simulink model "WSLS_X_Y_Rz3"  (R2025a)
settings: Solver=FixedStepAuto  StartTime=0.0  StopTime=t_end  FixedStep=0.0002  RelTol=1e-3  EnableMultiTasking=on
values from neighbouring files (symbols this model uses):
  rzQ = mz/k    (= 4.2809)    [Multiple_main_Control.m]
  Tb = pinv(B1)    [Multiple_main_Control.m]
  Ty = pinv(C1)    [Multiple_main_Control.m]
  xQ = Jrx/k    (= 0.0439)    [Multiple_main_Control.m]
  yQ = Jry/k    (= 0.0384)    [Multiple_main_Control.m]
undefined symbols (not defined in the file or in its folder): den_Cfb_rz, den_Cfb_x, den_Cfb_y, den_P11, den_P12, den_P13, den_P14, den_P21, den_P22, den_P23, den_P24, den_P31, den_P32, den_P33, den_P34, den_P41, den_P42, den_P43, den_P44, num_Cfb_rz, num_Cfb_x, num_Cfb_y, num_P11, num_P12, num_P13, num_P14, num_P21, num_P22, num_P23, num_P24, num_P31, num_P32, num_P33, num_P34, num_P41, num_P42, num_P43, num_P44
settings Model: Creator=zhang chen  LastModifiedBy=gdc24
settings DataIOCC: ReturnWorkspaceOutputs=off
settings OptimizationCC: ReuseModelBlockBuffer=off
settings DebuggingCC: UnconnectedInputMsg=warning  UnconnectedOutputMsg=warning  UnconnectedLineMsg=warning
settings ModelReferenceCC: EnableRefExpFcnMdlSchedulingChecks=on
settings RTWCC: GPUComputeCapability=3.5  DLArmComputeVersion=19.05

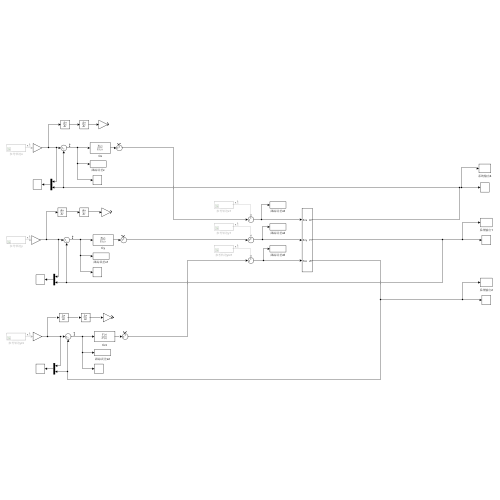
[thumbnail: Simulink's stored preview of the top-level diagram]
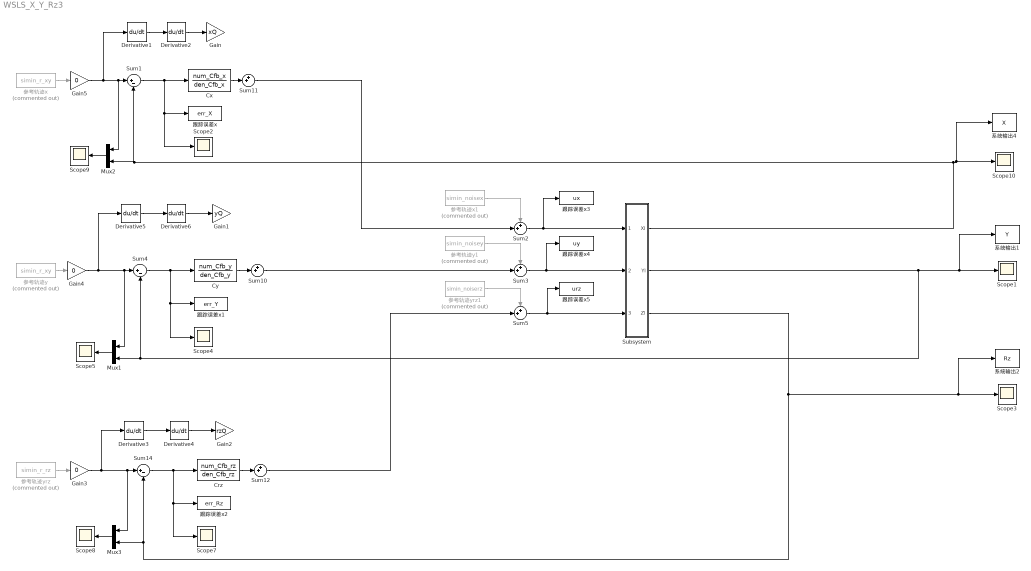
== system WSLS_X_Y_Rz3 ==
  Crz : TransferFcn  Numerator=num_Cfb_rz  Denominator=den_Cfb_rz
  Cx : TransferFcn  Numerator=num_Cfb_x  Denominator=den_Cfb_x
  Cy : TransferFcn  Numerator=num_Cfb_y  Denominator=den_Cfb_y
  Derivative{1..6} (6 alike) : Derivative
  Gain : Gain  Gain=xQ
  Gain1 : Gain  Gain=yQ
  Gain2 : Gain  Gain=rzQ
  Gain3 : Gain  Gain=0
  Gain4 : Gain  Gain=0
  Gain5 : Gain  Gain=0
  Mux1 : Mux  Inputs=2
  Mux2 : Mux  Inputs=2
  Mux3 : Mux  Inputs=2
  Scope{1..5,7..10} (9 alike) : Scope
      Scope1 settings: ActiveDisplayYMinimum=-8.79901930835965E-7  ActiveDisplayYMaximum=1.0139843335391608E-6  DataLoggingVariableName=ScopeData2
      Scope10 settings: ActiveDisplayYMinimum=-5.7566992518821054E-6  ActiveDisplayYMaximum=3.1982882643224368E-6
      Scope2 settings: ActiveDisplayYMinimum=-9E-7  ActiveDisplayYMaximum=9E-7
      Scope3 settings: ActiveDisplayYMinimum=-2.3040708038382956E-6  ActiveDisplayYMaximum=2.1091467969503966E-6  DataLoggingVariableName=ScopeData3
      Scope4 settings: ActiveDisplayYMinimum=-5E-7  ActiveDisplayYMaximum=6E-7  DataLoggingVariableName=ScopeData4
      Scope5 settings: ActiveDisplayYMinimum=-0.225  ActiveDisplayYMaximum=0.025  DataLoggingVariableName=ScopeData5
      Scope7 settings: ActiveDisplayYMinimum=-3.8E-5  ActiveDisplayYMaximum=3.8E-5  DataLoggingVariableName=ScopeData2
      Scope8 settings: ActiveDisplayYMinimum=-0.00111  ActiveDisplayYMaximum=0.01125  DataLoggingVariableName=ScopeData3
      Scope9 settings: ActiveDisplayYMinimum=-0.225  ActiveDisplayYMaximum=0.025  DataLoggingVariableName=ScopeData2
  Subsystem : Subsystem
  Sum1 : Sum  Inputs=|+-
  Sum{2..3,5,10..12} (6 alike) : Sum  Inputs=++|
  Sum14 : Sum  Inputs=|+-
  Sum4 : Sum  Inputs=|+-
  参考轨迹x : FromWorkspace  Commented=on  VariableName=simin_r_xy
  参考轨迹x1 : FromWorkspace  Commented=on  VariableName=simin_noisex
  参考轨迹y : FromWorkspace  Commented=on  VariableName=simin_r_xy
  参考轨迹y1 : FromWorkspace  Commented=on  VariableName=simin_noisey
  参考轨迹yrz : FromWorkspace  Commented=on  VariableName=simin_r_rz
  参考轨迹yrz1 : FromWorkspace  Commented=on  VariableName=simin_noiserz
  系统输出1 : ToWorkspace  VariableName=Y  SampleTime=-1
  系统输出2 : ToWorkspace  VariableName=Rz  SampleTime=-1
  系统输出4 : ToWorkspace  VariableName=X  SampleTime=-1
  跟踪误差x : ToWorkspace  VariableName=err_X  SampleTime=-1
  跟踪误差x1 : ToWorkspace  VariableName=err_Y  SampleTime=-1
  跟踪误差x2 : ToWorkspace  VariableName=err_Rz  SampleTime=-1
  跟踪误差x3 : ToWorkspace  VariableName=ux  SampleTime=-1
  跟踪误差x4 : ToWorkspace  VariableName=uy  SampleTime=-1
  跟踪误差x5 : ToWorkspace  VariableName=urz  SampleTime=-1
  wires:
  Sum1/1 -> Scope2/1, 跟踪误差x/1, Cx/1
  参考轨迹x/1 -> Gain5/1
  Mux2/1 -> Scope9/1
  Sum4/1 -> Scope4/1, 跟踪误差x1/1, Cy/1
  参考轨迹y/1 -> Gain4/1
  Mux1/1 -> Scope5/1
  Derivative5/1 -> Derivative6/1
  Cy/1 -> Sum10/2
  Derivative1/1 -> Derivative2/1
  Derivative2/1 -> Gain/1
  Cx/1 -> Sum11/2
  Crz/1 -> Sum12/2
  Mux3/1 -> Scope8/1
  Derivative3/1 -> Derivative4/1
  Derivative4/1 -> Gain2/1
  Sum14/1 -> Scope7/1, 跟踪误差x2/1, Crz/1
  参考轨迹yrz/1 -> Gain3/1
  Subsystem/1(Xl) -> 系统输出4/1, Scope10/1, Mux2/2, Sum1/2
  Subsystem/2(Yl) -> 系统输出1/1, Scope1/1, Mux1/2, Sum4/2
  Subsystem/3(Zl) -> 系统输出2/1, Scope3/1, Mux3/2, Sum14/2
  Derivative6/1 -> Gain1/1
  参考轨迹x1/1 -> Sum2/1
  Sum2/1 -> 跟踪误差x3/1, Subsystem/1(Fcx)
  Sum11/1 -> Sum2/2
  Sum3/1 -> 跟踪误差x4/1, Subsystem/2(Fcy)
  Sum10/1 -> Sum3/2
  Sum5/1 -> 跟踪误差x5/1, Subsystem/3(Tcz)
  Sum12/1 -> Sum5/2
  参考轨迹y1/1 -> Sum3/1
  参考轨迹yrz1/1 -> Sum5/1
  Gain3/1 -> Mux3/1, Sum14/1, Derivative3/1
  Gain4/1 -> Mux1/1, Sum4/1, Derivative5/1
  Gain5/1 -> Mux2/1, Sum1/1, Derivative1/1

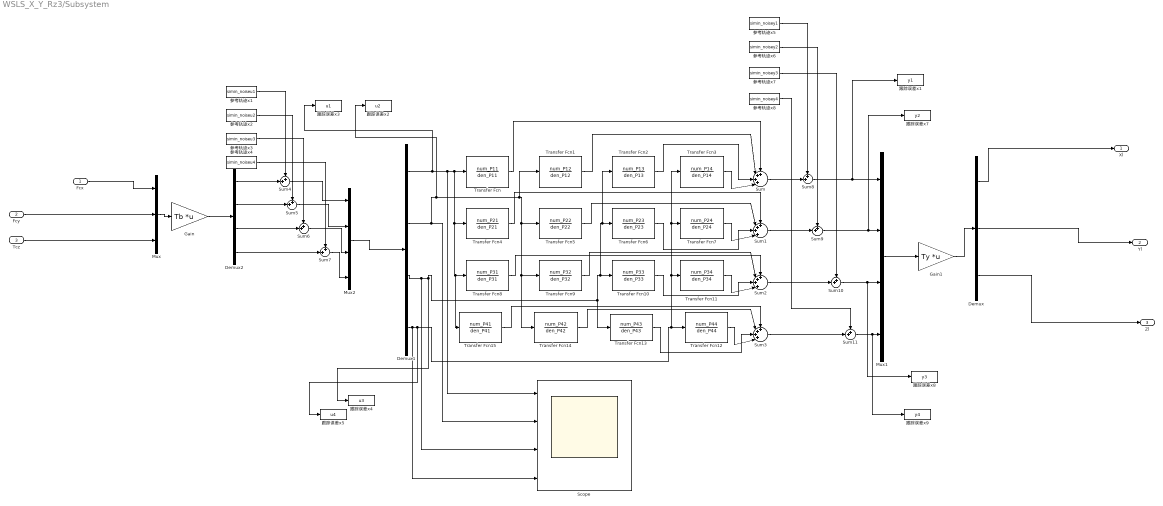
== system WSLS_X_Y_Rz3/Subsystem ==
  Fcx : Inport
  Fcy : Inport  Port=2
  Tcz : Inport  Port=3
  Demux : Demux  Outputs=3
  Demux1 : Demux
  Demux2 : Demux
  Gain : Gain  Gain=Tb  Multiplication=Matrix(K*u)
  Gain1 : Gain  Gain=Ty  Multiplication=Matrix(K*u)
  Mux : Mux  Inputs=3
  Mux1 : Mux
  Mux2 : Mux
  Scope : Scope  NumInputPorts=4
      settings: ActiveDisplayYMinimum=-7.6390835738538776  ActiveDisplayYMaximum=10.348276134391678  DataLoggingSaveFormat=Array
  Sum{,1..3} (4 alike) : Sum  Inputs=++++|
  Sum{4..11} (8 alike) : Sum  Inputs=++|
  Transfer Fcn : TransferFcn  Numerator=num_P11  Denominator=den_P11
  Transfer Fcn1 : TransferFcn  Numerator=num_P12  Denominator=den_P12
  Transfer Fcn10 : TransferFcn  Numerator=num_P33  Denominator=den_P33
  Transfer Fcn11 : TransferFcn  Numerator=num_P34  Denominator=den_P34
  Transfer Fcn12 : TransferFcn  Numerator=num_P44  Denominator=den_P44
  Transfer Fcn13 : TransferFcn  Numerator=num_P43  Denominator=den_P43
  Transfer Fcn14 : TransferFcn  Numerator=num_P42  Denominator=den_P42
  Transfer Fcn15 : TransferFcn  Numerator=num_P41  Denominator=den_P41
  Transfer Fcn2 : TransferFcn  Numerator=num_P13  Denominator=den_P13
  Transfer Fcn3 : TransferFcn  Numerator=num_P14  Denominator=den_P14
  Transfer Fcn4 : TransferFcn  Numerator=num_P21  Denominator=den_P21
  Transfer Fcn5 : TransferFcn  Numerator=num_P22  Denominator=den_P22
  Transfer Fcn6 : TransferFcn  Numerator=num_P23  Denominator=den_P23
  Transfer Fcn7 : TransferFcn  Numerator=num_P24  Denominator=den_P24
  Transfer Fcn8 : TransferFcn  Numerator=num_P31  Denominator=den_P31
  Transfer Fcn9 : TransferFcn  Numerator=num_P32  Denominator=den_P32
  参考轨迹x1 : FromWorkspace  VariableName=simin_noiseu1
  参考轨迹x2 : FromWorkspace  VariableName=simin_noiseu2
  参考轨迹x3 : FromWorkspace  VariableName=simin_noiseu3
  参考轨迹x4 : FromWorkspace  VariableName=simin_noiseu4
  参考轨迹x5 : FromWorkspace  VariableName=simin_noisey1
  参考轨迹x6 : FromWorkspace  VariableName=simin_noisey2
  参考轨迹x7 : FromWorkspace  VariableName=simin_noisey3
  参考轨迹x8 : FromWorkspace  VariableName=simin_noisey4
  跟踪误差x1 : ToWorkspace  VariableName=y1  SampleTime=-1
  跟踪误差x2 : ToWorkspace  VariableName=u2  SampleTime=-1
  跟踪误差x3 : ToWorkspace  VariableName=u1  SampleTime=-1
  跟踪误差x4 : ToWorkspace  VariableName=u3  SampleTime=-1
  跟踪误差x5 : ToWorkspace  VariableName=u4  SampleTime=-1
  跟踪误差x7 : ToWorkspace  VariableName=y2  SampleTime=-1
  跟踪误差x8 : ToWorkspace  VariableName=y3  SampleTime=-1
  跟踪误差x9 : ToWorkspace  VariableName=y4  SampleTime=-1
  Xl : Outport
  Yl : Outport  Port=2
  Zl : Outport  Port=3
  wires:
  Fcx/1 -> Mux/1
  Fcy/1 -> Mux/2
  Tcz/1 -> Mux/3
  Mux/1 -> Gain/1
  Gain1/1 -> Demux/1
  Demux/1 -> Xl/1
  Demux/2 -> Yl/1
  Demux/3 -> Zl/1
  Demux1/1 -> 跟踪误差x3/1, Scope/1, Transfer Fcn15/1, Transfer Fcn8/1, Transfer Fcn4/1, Transfer Fcn/1
  Demux1/2 -> Scope/2, 跟踪误差x2/1, Transfer Fcn1/1, Transfer Fcn14/1, Transfer Fcn9/1, Transfer Fcn5/1
  Demux1/3 -> Scope/3, Transfer Fcn10/1, Transfer Fcn2/1, Transfer Fcn6/1, Transfer Fcn13/1, 跟踪误差x4/1
  Demux1/4 -> Scope/4, 跟踪误差x5/1, Transfer Fcn3/1, Transfer Fcn7/1, Transfer Fcn11/1, Transfer Fcn12/1
  Transfer Fcn/1 -> Sum/1
  Transfer Fcn1/1 -> Sum/2
  Transfer Fcn2/1 -> Sum/3
  Transfer Fcn3/1 -> Sum/4
  Transfer Fcn4/1 -> Sum1/1
  Transfer Fcn5/1 -> Sum1/2
  Transfer Fcn6/1 -> Sum1/3
  Transfer Fcn7/1 -> Sum1/4
  Transfer Fcn8/1 -> Sum2/1
  Transfer Fcn9/1 -> Sum2/2
  Transfer Fcn10/1 -> Sum2/3
  Transfer Fcn11/1 -> Sum2/4
  Transfer Fcn15/1 -> Sum3/1
  Transfer Fcn14/1 -> Sum3/2
  Transfer Fcn13/1 -> Sum3/3
  Transfer Fcn12/1 -> Sum3/4
  Gain/1 -> Demux2/1
  Mux2/1 -> Demux1/1
  Demux2/1 -> Sum4/2
  Demux2/2 -> Sum5/2
  Demux2/3 -> Sum6/2
  Demux2/4 -> Sum7/2
  Sum7/1 -> Mux2/4
  Sum6/1 -> Mux2/3
  Sum5/1 -> Mux2/2
  Sum4/1 -> Mux2/1
  参考轨迹x1/1 -> Sum4/1
  参考轨迹x2/1 -> Sum5/1
  参考轨迹x3/1 -> Sum6/1
  参考轨迹x4/1 -> Sum7/1
  Mux1/1 -> Gain1/1
  Sum/1 -> Sum8/2
  Sum8/1 -> 跟踪误差x1/1, Mux1/1
  Sum1/1 -> Sum9/2
  Sum9/1 -> 跟踪误差x7/1, Mux1/2
  Sum2/1 -> Sum10/2
  Sum10/1 -> Mux1/3, 跟踪误差x8/1
  Sum11/1 -> 跟踪误差x9/1, Mux1/4
  Sum3/1 -> Sum11/2
  参考轨迹x5/1 -> Sum8/1
  参考轨迹x6/1 -> Sum9/1
  参考轨迹x7/1 -> Sum10/1
  参考轨迹x8/1 -> Sum11/1
